simulink subsystem "piero_model"  (R2022b)
settings: Solver=VariableStepAuto  StartTime=0.0  StopTime=10.0  RelTol=1e-3
settings Model: Creator=miriamfreiriasanjuan  LastModifiedBy=miriamfreiriasanjuan

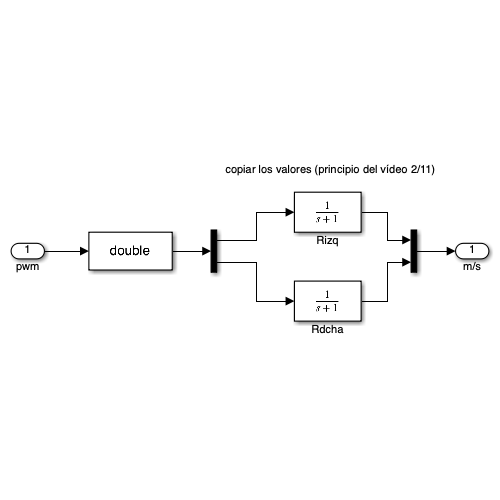
[thumbnail: Simulink's stored preview of the top-level diagram]
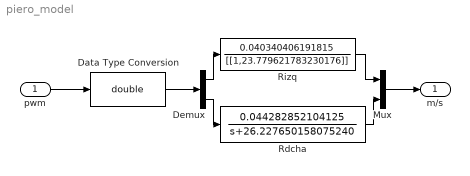
== system piero_model ==
  pwm : Inport
  Data Type Conversion : DataTypeConversion  OutDataTypeStr=double  SaturateOnIntegerOverflow=off  RndMeth=Floor
  Demux : Demux  Outputs=2
  Mux : Mux  Inputs=2
  Rdcha : TransferFcn  Numerator=[0.044282852104125]  Denominator=[1,26.227650158075240]
  Rizq : TransferFcn  Numerator=[0.040340406191815]  Denominator=[[1,23.779621783230176]]
  m/s : Outport
  wires:
  pwm/1 -> Data Type Conversion/1
  Mux/1 -> m/s/1
  Demux/1 -> Rizq/1
  Demux/2 -> Rdcha/1
  Rizq/1 -> Mux/1
  Rdcha/1 -> Mux/2
  Data Type Conversion/1 -> Demux/1
